simulink model "simulin8"  (R2022b)
settings: Solver=VariableStepAuto  StartTime=0.0  StopTime=1  RelTol=1e-3
values from neighbouring files (symbols this model uses):
  An = A-B*k    [M8.m]
  B = [0 ; 61.065 ; 0 ; -61.065]    [M8.m]
  C = [1 0 0 0]    [M8.m]
settings Model: Creator=ali14  LastModifiedBy=ali14

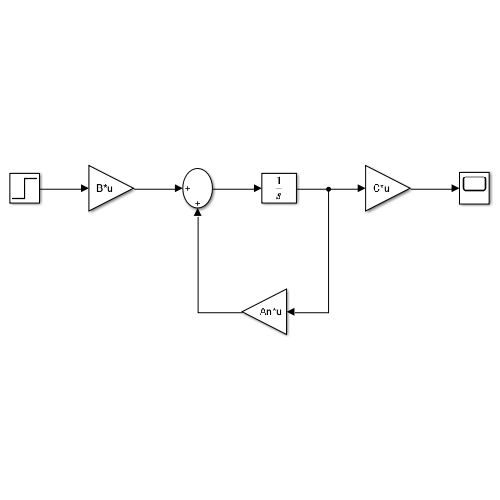
[thumbnail: Simulink's stored preview of the top-level diagram]
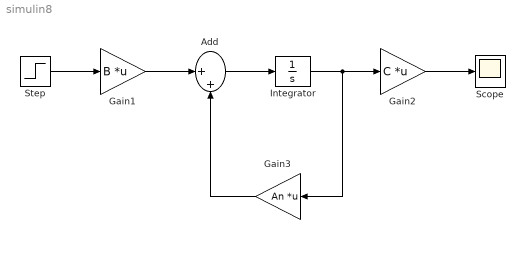
== system simulin8 ==
  Add : Sum  Inputs=|++
  Gain1 : Gain  Gain=B  Multiplication=Matrix(K*u)
  Gain2 : Gain  Gain=C  Multiplication=Matrix(K*u)
  Gain3 : Gain  Gain=An  Multiplication=Matrix(K*u)
  Integrator : Integrator  InitialCondition=zeros(4,1)
  Scope : Scope
  Step : Step  Time=0  SampleTime=0
  wires:
  Add/1 -> Integrator/1
  Integrator/1 -> Gain2/1, Gain3/1
  Gain2/1 -> Scope/1
  Gain3/1 -> Add/2
  Gain1/1 -> Add/1
  Step/1 -> Gain1/1
